simulink model "Final"  (R2023b)
settings: Solver=VariableStepAuto  StartTime=0.0  StopTime=150  FixedStep=0.05  RelTol=1e-5
undefined symbols (not defined in the file): adapt, ctrl, k_f, MRAC_on, Omega_prop_0, omegab_0, p_i_0, package_exist, par, pb_gate_cfg, q_0, robust_on, T_prop_0, task4_ground_z, UAV, UAV_pkg, v_i_0, vb_0
libraries: aerolibutil x3, sharedtransform x2, simulink_extras x2
settings Model: Creator=justs  LastModifiedBy=mghor
settings SolverCC: ZeroCrossAlgorithm=Adaptive
settings DataIOCC: SaveOutput=off  SignalLogging=off
settings OptimizationCC: ReuseModelBlockBuffer=off
settings DebuggingCC: IgnoredZcDiagnostic=none
settings ModelReferenceCC: EnableRefExpFcnMdlSchedulingChecks=on
settings ConfigComp: CovBoundaryAbsTol=1.0e-5

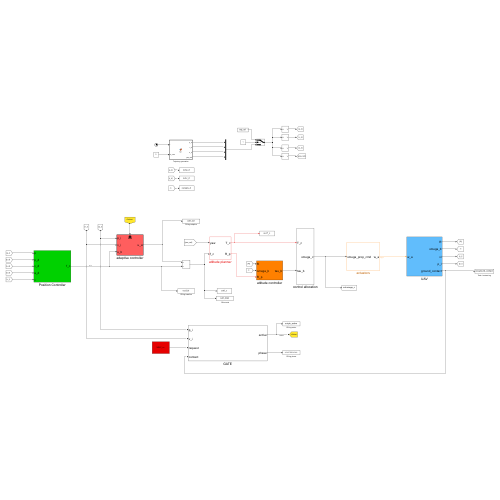
[thumbnail: Simulink's stored preview of the top-level diagram]
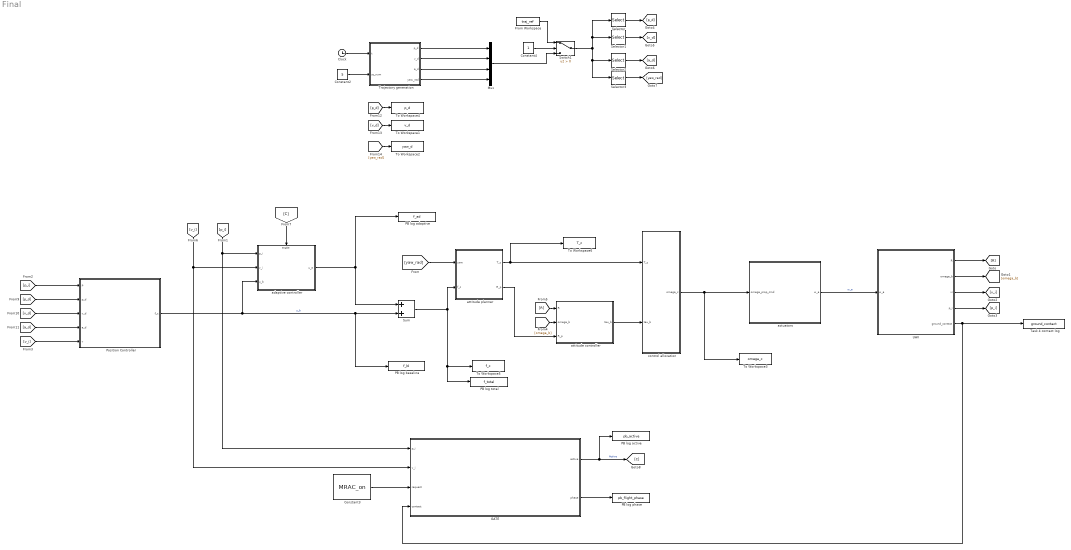
== system Final ==
  Clock : Clock
  Constant2 : Constant  Value=5
  Constant3 : Constant  Value=MRAC_on
  Constant4 : Constant
  From Workspace : FromWorkspace  VariableName=traj_ref  ZeroCross=off
  GATE : Subsystem
  Mux : Mux
  PB log active : ToWorkspace  VariableName=pb_active  SaveFormat=Timeseries  SampleTime=-1
  PB log adaptive : ToWorkspace  VariableName=f_ad  SaveFormat=Timeseries  SampleTime=-1
  PB log baseline : ToWorkspace  VariableName=f_bl  SaveFormat=Timeseries  SampleTime=-1
  PB log phase : ToWorkspace  VariableName=pb_flight_phase  SaveFormat=Timeseries  SampleTime=-1
  PB log total : ToWorkspace  VariableName=f_total  SaveFormat=Timeseries  SampleTime=-1
  Position Controller : Subsystem
  Selector : Selector  InputPortWidth=10  IndexOptions=Index vector (dialog)  Indices=[1 2 3]  OutputSizes=1
  Selector1 : Selector  InputPortWidth=10  IndexOptions=Index vector (dialog)  Indices=[4 5 6]  OutputSizes=1
  Selector2 : Selector  InputPortWidth=10  IndexOptions=Index vector (dialog)  Indices=[7 8 9]  OutputSizes=1
  Selector3 : Selector  InputPortWidth=10  IndexOptions=Index vector (dialog)  Indices=[10]  OutputSizes=1
  Sum : Sum
  Switch1 : Switch  Criteria=u2 > Threshold  SaturateOnIntegerOverflow=off  InputSameDT=off
  Task 4 contact log : ToWorkspace  VariableName=ground_contact  SaveFormat=Timeseries  SampleTime=-1
  To Workspace1 : ToWorkspace  VariableName=v_d  SaveFormat=Timeseries  SampleTime=-1
  To Workspace2 : ToWorkspace  VariableName=yaw_d  SaveFormat=Timeseries  SampleTime=-1
  To Workspace3 : ToWorkspace  VariableName=omega_c  SaveFormat=Timeseries  SampleTime=-1
  To Workspace4 : ToWorkspace  VariableName=p_d  SaveFormat=Timeseries  SampleTime=-1
  To Workspace5 : ToWorkspace  VariableName=f_c  SaveFormat=Timeseries  SampleTime=-1
  To Workspace6 : ToWorkspace  VariableName=T_c  SaveFormat=Timeseries  SampleTime=-1
  Trajectory generation : MATLAB Function  TreatAsAtomicUnit=on
  UAV : Subsystem
  actuators : Subsystem
  adaptive controller : Subsystem
  attitude controller : Subsystem
  attitude planner : Subsystem
  control allocation : Subsystem
  wires:
  Trajectory generation/2(v_d) -> Mux/2
  Trajectory generation/3(a_d) -> Mux/3
  Trajectory generation/1(p_d) -> Mux/1
  Clock/1 -> Trajectory generation/1(t)
  [p_i] -> Position Controller/1(p)
  [v_i] -> Position Controller/5(v)
  attitude planner/2(R_p) -> attitude controller/3(R_p)
  [omega_b] -> attitude controller/2(omega_b)
  [R] -> attitude controller/1(R)
  attitude planner/1(T_c) -> To Workspace6/1, control allocation/1(T_c)
  attitude controller/1(tau_b) -> control allocation/2(tau_b)
  control allocation/1(omega_c) -> To Workspace3/1, actuators/1(omega_prop_cmd)
  Trajectory generation/4(yaw_rad) -> Mux/4
  UAV/1(R) -> [R]
  UAV/2(omega_b) -> [omega_b]
  UAV/3(vi) -> [v_i]
  UAV/4(p_i) -> [p_i]
  Constant2/1 -> Trajectory generation/2(sc_num)
  actuators/1(w_a) -> UAV/1(w_a)  "w_a"
  [p_i] -> GATE/1(p_i), adaptive controller/1(p_i)
  [v_i] -> adaptive controller/2(v_i), GATE/2(v_i)
  Sum/1 -> PB log total/1, To Workspace5/1, attitude planner/2(f_c)
  Mux/1 -> Switch1/3
  Constant4/1 -> Switch1/2
  From Workspace/1 -> Switch1/1
  Selector/1 -> [p_d]
  Selector1/1 -> [v_d]
  Selector2/1 -> [a_d]
  Selector3/1 -> [yaw_rad]
  [yaw_rad] -> attitude planner/1(yaw)
  [p_d] -> Position Controller/2(p_d)
  [v_d] -> Position Controller/3(v_d)
  [a_d] -> Position Controller/4(a_d)
  [p_d] -> To Workspace4/1
  [v_d] -> To Workspace1/1
  [yaw_rad] -> To Workspace2/1
  Position Controller/1(f_c) -> Sum/2, PB log baseline/1, adaptive controller/3(u_b)  "u_b"
  adaptive controller/1(" u_a") -> PB log adaptive/1, Sum/1
  Switch1/1 -> Selector2/1, Selector3/1, Selector1/1, Selector/1
  UAV/5(ground_contact) -> GATE/4(contact), Task 4 contact log/1
  GATE/1(active) -> [C], PB log active/1  "Active"
  Constant3/1 -> GATE/3(request)
  GATE/2(phase) -> PB log phase/1
  [C] -> adaptive controller/Enable

== system Final/GATE ==
  p_i : Inport
  v_i : Inport  Port=2
  request : Inport  Port=3
  contact : Inport  Port=4
  PBMRAC enable : Subsystem  Variant=on
  active : Outport
  phase : Outport  Port=2
  wires:
  PBMRAC enable/1(active) -> active/1
  p_i/1 -> PBMRAC enable/1(p_i)
  request/1 -> PBMRAC enable/3(request)
  PBMRAC enable/2(phase) -> phase/1
  v_i/1 -> PBMRAC enable/2(v_i)
  contact/1 -> PBMRAC enable/4(contact)

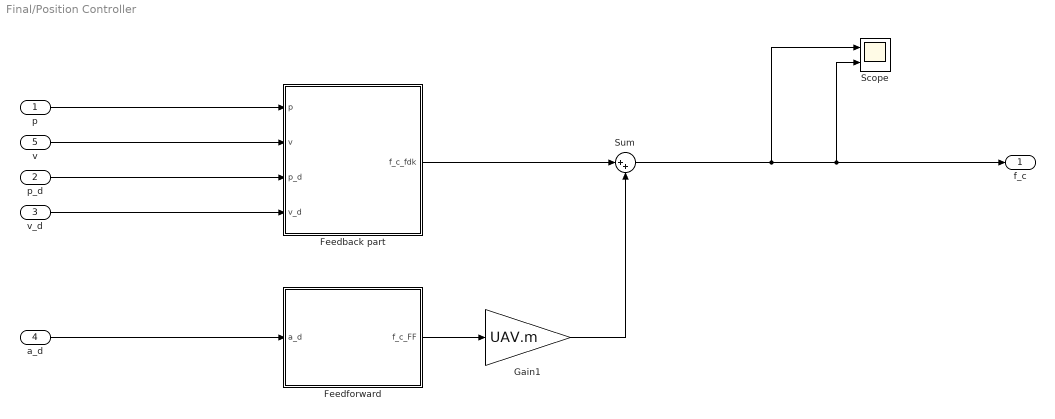
== system Final/Position Controller ==
  p : Inport
  p_d : Inport  Port=2
  v_d : Inport  Port=3
  a_d : Inport  Port=4
  v : Inport  Port=5
  Feedback part : Subsystem
  Feedforward : Subsystem
  Gain1 : Gain  Gain=UAV.m
  Scope : Scope  NumInputPorts=2
  Sum : Sum  Inputs=|++
  f_c : Outport
  wires:
  Feedback part/1(f_c_fdk) -> Sum/1
  v_d/1 -> Feedback part/4(v_d)
  Feedforward/1(f_c_FF) -> Gain1/1
  a_d/1 -> Feedforward/1(a_d)
  v/1 -> Feedback part/2(v)
  p_d/1 -> Feedback part/3(p_d)
  p/1 -> Feedback part/1(p)
  Sum/1 -> f_c/1, Scope/2, Scope/1
  Gain1/1 -> Sum/2

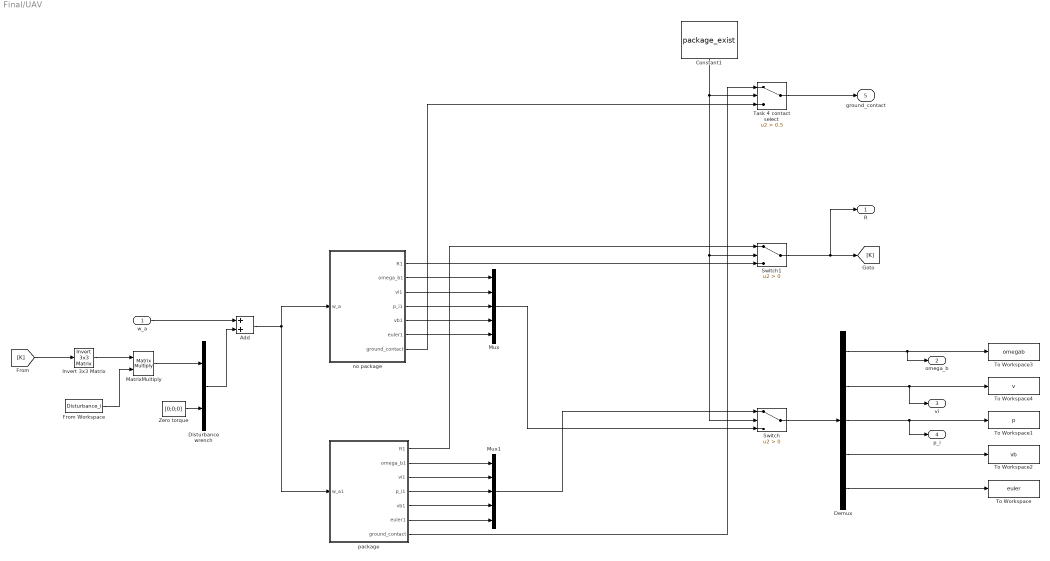
== system Final/UAV ==
  w_a : Inport
  Add : Sum
  Constant1 : Constant  Value=package_exist
  Demux : Demux  Outputs=5
  Disturbance wrench : Mux  Inputs=2
  From Workspace : FromWorkspace  VariableName=Disturbance_i
  Invert 3x3 Matrix : aerolibutil/Invert  3x3 Matrix
  MatrixMultiply : Product  Multiplication=Matrix(*)
  Mux : Mux  Inputs=5
  Mux1 : Mux  Inputs=5
  Switch : Switch  Criteria=u2 > Threshold  SaturateOnIntegerOverflow=off  InputSameDT=off
  Switch1 : Switch  Criteria=u2 > Threshold  SaturateOnIntegerOverflow=off  InputSameDT=off
  Task 4 contact select : Switch  Criteria=u2 > Threshold  Threshold=0.5  SaturateOnIntegerOverflow=off  InputSameDT=off
  To Workspace : ToWorkspace  VariableName=euler  SaveFormat=Timeseries  SampleTime=-1
  To Workspace1 : ToWorkspace  VariableName=p  SaveFormat=Timeseries  SampleTime=-1
  To Workspace2 : ToWorkspace  VariableName=vb  SaveFormat=Timeseries  SampleTime=-1
  To Workspace3 : ToWorkspace  VariableName=omegab  SaveFormat=Timeseries  SampleTime=-1
  To Workspace4 : ToWorkspace  VariableName=v  SaveFormat=Timeseries  SampleTime=-1
  Zero torque : Constant  Value=[0;0;0]
  no package : Subsystem
  package : Subsystem
  R : Outport
  omega_b : Outport  Port=2
  vi : Outport  Port=3
  p_i : Outport  Port=4
  ground_contact : Outport  Port=5
  wires:
  Constant1/1 -> Switch/2, Switch1/2, Task 4 contact select/2
  Mux1/1 -> Switch/1
  Mux/1 -> Switch/3
  no package/2(omega_b1) -> Mux/1
  no package/3(vi1) -> Mux/2
  no package/4(p_i1) -> Mux/3
  no package/5(vb1) -> Mux/4
  no package/6(euler1) -> Mux/5
  package/2(omega_b1) -> Mux1/1
  package/3(vi1) -> Mux1/2
  package/4(p_i1) -> Mux1/3
  package/5(vb1) -> Mux1/4
  package/6(euler1) -> Mux1/5
  Switch/1 -> Demux/1
  Demux/1 -> omega_b/1, To Workspace3/1
  Demux/2 -> To Workspace4/1, vi/1
  Demux/3 -> To Workspace1/1, p_i/1
  Demux/4 -> To Workspace2/1
  Demux/5 -> To Workspace/1
  no package/1(R1) -> Switch1/3
  package/1(R1) -> Switch1/1
  From Workspace/1 -> MatrixMultiply/2
  Switch1/1 -> R/1, [K]
  Zero torque/1 -> Disturbance wrench/2
  Disturbance wrench/1 -> Add/2
  Invert 3x3 Matrix/1 -> MatrixMultiply/1
  MatrixMultiply/1 -> Disturbance wrench/1
  w_a/1 -> Add/1
  Add/1 -> no package/1(w_a), package/1(w_a1)
  package/7(ground_contact) -> Task 4 contact select/1
  no package/7(ground_contact) -> Task 4 contact select/3
  Task 4 contact select/1 -> ground_contact/1
  [K] -> Invert 3x3 Matrix/1

== system Final/actuators ==
  omega_prop_cmd : Inport
  Constant1 : Constant  Value=UAV.F2
  Constant2 : Constant  Value=UAV.F1
  MatrixMultiply1 : Product  Inputs=3  Multiplication=Matrix(*)
  To Workspace1 : ToWorkspace  VariableName=w_a  SaveFormat=Timeseries  SampleTime=-1
  To Workspace6 : ToWorkspace  VariableName=T_out  SaveFormat=Timeseries  SampleTime=-1
  rotor_speed : Subsystem
  thrust : Subsystem
  w_a : Outport
  wires:
  rotor_speed/1(omega_prop) -> thrust/1(omega_prop)
  Constant2/1 -> MatrixMultiply1/1
  thrust/1(thrust) -> MatrixMultiply1/3, To Workspace6/1
  omega_prop_cmd/1 -> rotor_speed/1(omega_prop_cmd)
  MatrixMultiply1/1 -> w_a/1, To Workspace1/1
  Constant1/1 -> MatrixMultiply1/2

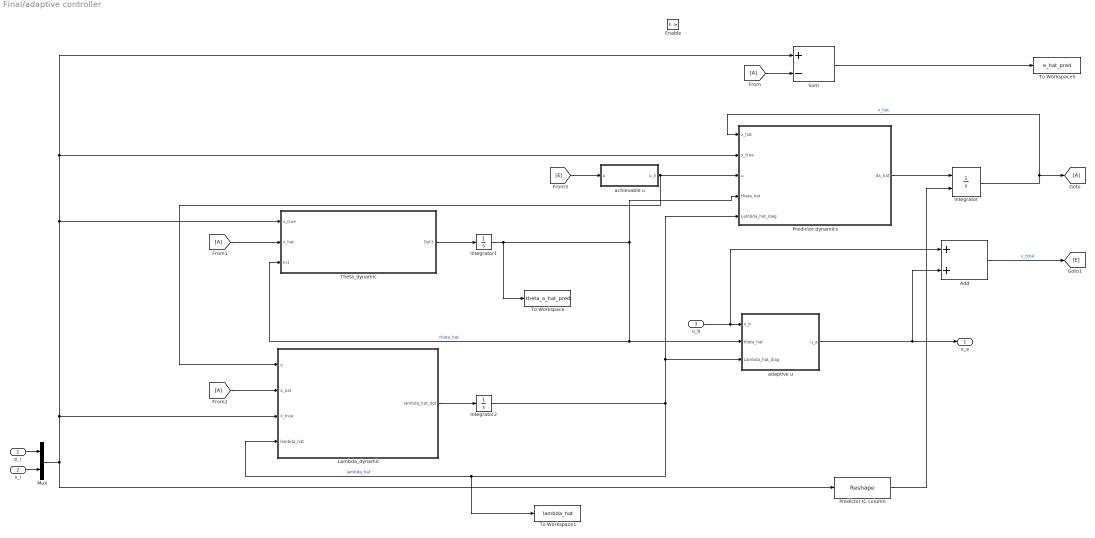
== system Final/adaptive controller ==
  p_i : Inport
  v_i : Inport  Port=2
  u_b : Inport  Port=3
  Enable : EnablePort  StatesWhenEnabling=reset
  Add : Sum
  From : From
  From1 : From
  From2 : From
  Goto : Goto
  Integrator : Integrator  InitialConditionSource=external  InitialCondition=[p_i_0; v_i_0]
  Integrator1 : Integrator  InitialCondition=[0; 0; 0]
  Integrator2 : Integrator  InitialCondition=[1;1;1]
  Lambda_dynamic : Subsystem
  Mux : Mux  Inputs=2
  Predictor IC column : Reshape  OutputDimensionality=Customize  OutputDimensions=[6 1]
  Predictor dynamics : MATLAB Function  TreatAsAtomicUnit=on
  Sum : Sum  Inputs=+-
  Theta_dynamic : Subsystem
  To Workspace : ToWorkspace  VariableName=theta_a_hat_pred  SaveFormat=Timeseries  SampleTime=-1
  To Workspace1 : ToWorkspace  VariableName=lambda_hat  SaveFormat=Timeseries  SampleTime=-1
  To Workspace5 : ToWorkspace  VariableName=e_hat_pred  SaveFormat=Timeseries  SampleTime=-1
  achievable u : MATLAB Function  TreatAsAtomicUnit=on
  adaptive u : MATLAB Function  TreatAsAtomicUnit=on
  " u_a" : Outport  OutputWhenDisabled=reset  InitialOutput=[0;0;0]
  wires:
  u_b/1 -> adaptive u/1(u_b), Add/1
  Add/1 -> [E]  "u_total"
  Integrator/1 -> Goto/1, Predictor dynamics/1(x_hat)  "x_hat"
  Integrator1/1 -> Predictor dynamics/4(theta_hat), Theta_dynamic/3(In1), adaptive u/2(theta_hat), To Workspace/1  "theta_hat"
  Integrator2/1 -> adaptive u/3(Lambda_hat_diag), Predictor dynamics/5(Lambda_hat_diag), To Workspace1/1, Lambda_dynamic/4(lambda_hat)  "lambda_hat"
  Mux/1 -> Sum/1, Predictor dynamics/2(x_true), Theta_dynamic/1(x_true), Lambda_dynamic/3(x_true), Predictor IC column/1
  adaptive u/1(u_a) -> " u_a"/1, Add/2
  From2/1 -> Lambda_dynamic/2(x_hat)
  From1/1 -> Theta_dynamic/2(x_hat)
  From/1 -> Sum/2
  Sum/1 -> To Workspace5/1
  Predictor dynamics/1(dx_hat) -> Integrator/1
  Theta_dynamic/1(Out1) -> Integrator1/1
  Lambda_dynamic/1(lambda_hat_dot) -> Integrator2/1
  p_i/1 -> Mux/1
  v_i/1 -> Mux/2
  achievable u/1(u_h) -> Predictor dynamics/3(u), Lambda_dynamic/1(u)
  Predictor IC column/1 -> Integrator/2
  [E] -> achievable u/1(u)

== system Final/attitude controller ==
  R : Inport
  omega_b : Inport  Port=2
  R_p : Inport  Port=3
  Gain : Gain  Gain=ctrl.Komega  Multiplication=Matrix(K*u)
  Saturation : Saturate  UpperLimit=1.2  LowerLimit=-1.2
  Scope : Scope  NumInputPorts=2
  Sum : Sum  Inputs=--
  e_R : MATLAB Function  TreatAsAtomicUnit=on
  tau_b : Outport
  wires:
  Saturation/1 -> Scope/2, tau_b/1
  e_R/1(e_R) -> Sum/1
  Sum/1 -> Saturation/1, Scope/1
  Gain/1 -> Sum/2
  R_p/1 -> e_R/2(R_d)
  R/1 -> e_R/1(R)
  omega_b/1 -> Gain/1

== system Final/attitude planner ==
  yaw : Inport
  f_c : Inport  Port=2
  MATLAB Function : MATLAB Function  TreatAsAtomicUnit=on
  T_c : Outport
  R_p : Outport  Port=2
  wires:
  yaw/1 -> MATLAB Function/1(yaw)
  f_c/1 -> MATLAB Function/2(f_c)
  MATLAB Function/1(T_c) -> T_c/1
  MATLAB Function/2(R_p) -> R_p/1

== system Final/control allocation ==
  T_c : Inport
  tau_b : Inport  Port=2
  Constant : Constant  Value=UAV.F2_pinv
  Constant1 : Constant  Value=k_f
  MATLAB Function : MATLAB Function  TreatAsAtomicUnit=on
  MATLAB Function1 : MATLAB Function  TreatAsAtomicUnit=on
  omega_c : Outport
  wires:
  T_c/1 -> MATLAB Function/1(T_c)
  tau_b/1 -> MATLAB Function/2(tau_b)
  MATLAB Function/1(Uc) -> MATLAB Function1/1(Uc)
  Constant/1 -> MATLAB Function/3(F2_pinv)
  MATLAB Function1/1(Omega_cmd) -> omega_c/1
  Constant1/1 -> MATLAB Function1/2(k_f)

== system Final/GATE/PBMRAC enable ==
  note: 1) Add Subsystem or Model blocks as valid variant choices.
      | 2) You cannot connect blocks at this level. At simulation, connectivity is automatically
      | determined, based on the active variant and port name matching.
  p_i : Inport
  v_i : Inport  Port=2
  request : Inport  Port=3
  contact : Inport  Port=4
  Direct : Subsystem  VariantControl=pb_flight_gate == 0
  Flight gate : Subsystem  VariantControl=pb_flight_gate == 1
  Subsystem1 : Subsystem  VariantControl=false
  active : Outport
  phase : Outport  Port=2

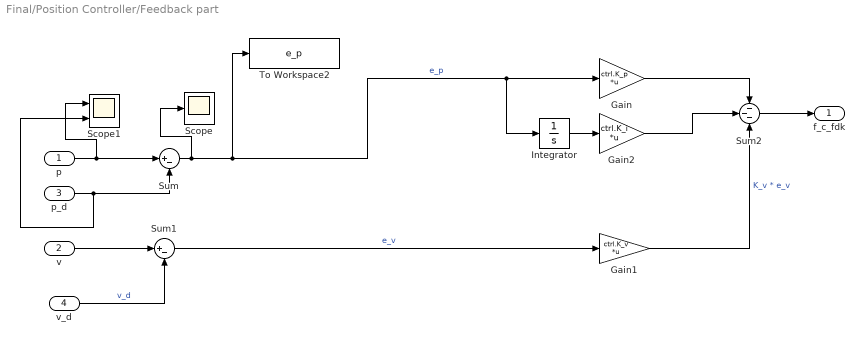
== system Final/Position Controller/Feedback part ==
  p : Inport
  v : Inport  Port=2
  p_d : Inport  Port=3
  v_d : Inport  Port=4
  Gain : Gain  Gain=ctrl.K_p  Multiplication=Matrix(K*u)
  Gain1 : Gain  Gain=ctrl.K_v  Multiplication=Matrix(K*u)
  Gain2 : Gain  Gain=ctrl.K_i  Multiplication=Matrix(K*u)
  Integrator : Integrator
  Scope : Scope
  Scope1 : Scope  NumInputPorts=2
  Sum : Sum  Inputs=|+-
  Sum1 : Sum  Inputs=|+-
  Sum2 : Sum  Inputs=---
  To Workspace2 : ToWorkspace  VariableName=e_p  SaveFormat=Timeseries  SampleTime=-1
  f_c_fdk : Outport
  wires:
  p_d/1 -> Scope1/2, Sum/2
  v/1 -> Sum1/1
  Sum1/1 -> Gain1/1  "e_v"
  v_d/1 -> Sum1/2  "v_d"
  p/1 -> Scope1/1, Sum/1
  Gain/1 -> Sum2/1
  Sum/1 -> Scope/1, To Workspace2/1, Integrator/1, Gain/1  "e_p"
  Integrator/1 -> Gain2/1
  Gain1/1 -> Sum2/3  "K_v * e_v"
  Sum2/1 -> f_c_fdk/1
  Gain2/1 -> Sum2/2

== system Final/Position Controller/Feedforward ==
  a_d : Inport
  Constant : Constant  Value=par.g*par.e_3
  Sum3 : Sum
  f_c_FF : Outport
  wires:
  Constant/1 -> Sum3/1
  a_d/1 -> Sum3/2
  Sum3/1 -> f_c_FF/1

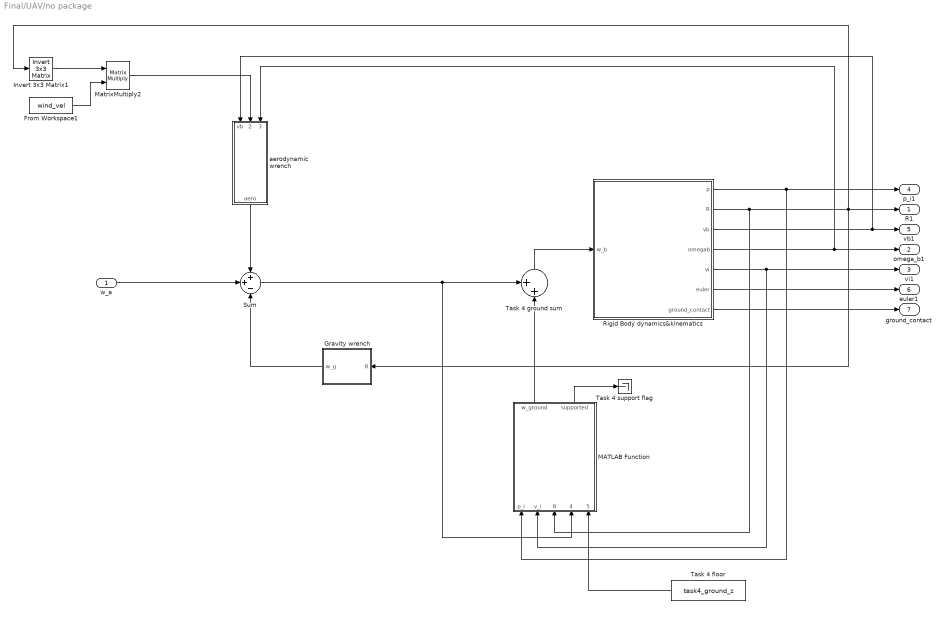
== system Final/UAV/no package ==
  w_a : Inport
  From Workspace1 : FromWorkspace  VariableName=wind_vel
  Gravity wrench : MATLAB Function  TreatAsAtomicUnit=on
  Invert 3x3 Matrix1 : aerolibutil/Invert  3x3 Matrix
  MATLAB Function : MATLAB Function  TreatAsAtomicUnit=on
  MatrixMultiply2 : Product  Multiplication=Matrix(*)
  "Rigid Body dynamics&kinematics " : Subsystem
  Sum : Sum  Inputs=++-
  Task 4 floor : Constant  Value=task4_ground_z
  Task 4 ground sum : Sum  Inputs=++|
  Task 4 support flag : Terminator
  aerodynamic wrench : Subsystem
  R1 : Outport
  omega_b1 : Outport  Port=2  PortDimensions=[3 1]
  vi1 : Outport  Port=3  PortDimensions=[3 1]
  p_i1 : Outport  Port=4  PortDimensions=[3 1]
  vb1 : Outport  Port=5  PortDimensions=[3 1]
  euler1 : Outport  Port=6  PortDimensions=[3 1]
  ground_contact : Outport  Port=7
  wires:
  "Rigid Body dynamics&kinematics "/4(omegab) -> omega_b1/1, aerodynamic wrench/3(omegab)
  "Rigid Body dynamics&kinematics "/3(vb) -> aerodynamic wrench/1(vb), vb1/1
  "Rigid Body dynamics&kinematics "/1(p) -> p_i1/1, MATLAB Function/1(p_i)
  "Rigid Body dynamics&kinematics "/5(vi) -> vi1/1, MATLAB Function/2(v_i)
  "Rigid Body dynamics&kinematics "/6(euler) -> euler1/1
  "Rigid Body dynamics&kinematics "/2(R) -> R1/1, Gravity wrench/1(R), Invert 3x3 Matrix1/1, MATLAB Function/3(R)
  aerodynamic wrench/1(aero) -> Sum/1
  Invert 3x3 Matrix1/1 -> MatrixMultiply2/1
  From Workspace1/1 -> MatrixMultiply2/2
  MatrixMultiply2/1 -> aerodynamic wrench/2(wind)
  Sum/1 -> MATLAB Function/4(w_free), Task 4 ground sum/1
  Task 4 ground sum/1 -> "Rigid Body dynamics&kinematics "/1(w_b)
  MATLAB Function/2(supported) -> Task 4 support flag/1
  "Rigid Body dynamics&kinematics "/7(ground_contact) -> ground_contact/1
  Task 4 floor/1 -> MATLAB Function/5(ground_z)
  w_a/1 -> Sum/2
  Gravity wrench/1(w_g) -> Sum/3
  MATLAB Function/1(w_ground) -> Task 4 ground sum/2

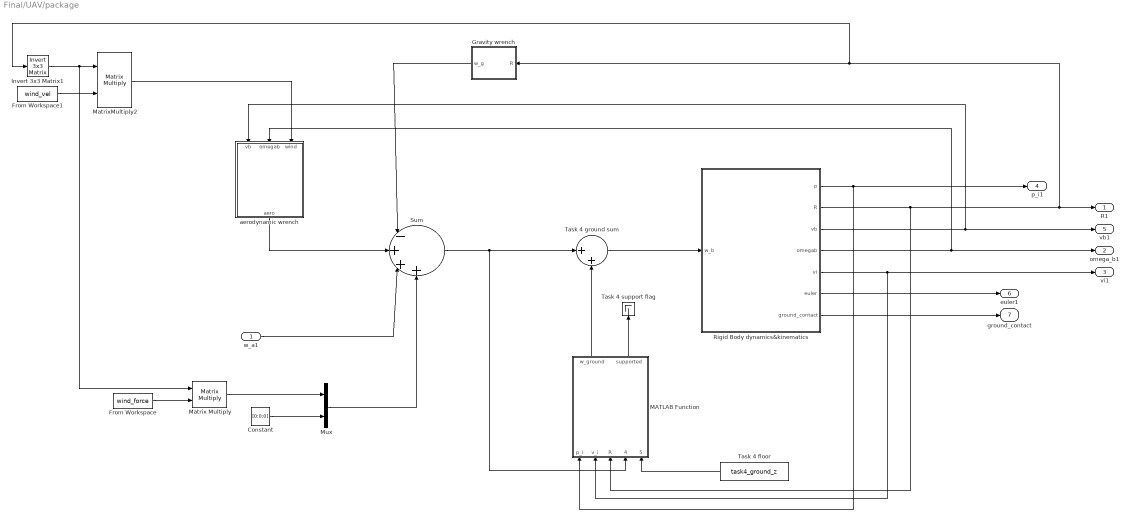
== system Final/UAV/package ==
  w_a1 : Inport
  Constant : Constant  Value=[0;0;0]
  From Workspace : FromWorkspace  VariableName=wind_force
  From Workspace1 : FromWorkspace  VariableName=wind_vel
  Gravity wrench : MATLAB Function  TreatAsAtomicUnit=on
  Invert 3x3 Matrix1 : aerolibutil/Invert  3x3 Matrix
  MATLAB Function : MATLAB Function  TreatAsAtomicUnit=on
  Matrix Multiply : Product  Multiplication=Matrix(*)
  MatrixMultiply2 : Product  Multiplication=Matrix(*)
  Mux : Mux  Inputs=2
  "Rigid Body dynamics&kinematics " : Subsystem
  Sum : Sum  Inputs=|-+++
  Task 4 floor : Constant  Value=task4_ground_z
  Task 4 ground sum : Sum  Inputs=|++
  Task 4 support flag : Terminator
  aerodynamic wrench : Subsystem
  R1 : Outport
  omega_b1 : Outport  Port=2  PortDimensions=[3 1]
  vi1 : Outport  Port=3  PortDimensions=[3 1]
  p_i1 : Outport  Port=4  PortDimensions=[3 1]
  vb1 : Outport  Port=5  PortDimensions=[3 1]
  euler1 : Outport  Port=6  PortDimensions=[3 1]
  ground_contact : Outport  Port=7
  wires:
  "Rigid Body dynamics&kinematics "/1(p) -> p_i1/1, MATLAB Function/1(p_i)
  "Rigid Body dynamics&kinematics "/5(vi) -> vi1/1, MATLAB Function/2(v_i)
  w_a1/1 -> Sum/3
  "Rigid Body dynamics&kinematics "/3(vb) -> vb1/1, aerodynamic wrench/1(vb)
  "Rigid Body dynamics&kinematics "/2(R) -> Invert 3x3 Matrix1/1, Gravity wrench/1(R), R1/1, MATLAB Function/3(R)
  "Rigid Body dynamics&kinematics "/4(omegab) -> omega_b1/1, aerodynamic wrench/2(omegab)
  "Rigid Body dynamics&kinematics "/6(euler) -> euler1/1
  aerodynamic wrench/1(aero) -> Sum/2
  Invert 3x3 Matrix1/1 -> Matrix Multiply/1, MatrixMultiply2/1
  From Workspace1/1 -> MatrixMultiply2/2
  MatrixMultiply2/1 -> aerodynamic wrench/3(wind)
  Gravity wrench/1(w_g) -> Sum/1
  From Workspace/1 -> Matrix Multiply/2
  Matrix Multiply/1 -> Mux/1
  Constant/1 -> Mux/2
  Mux/1 -> Sum/4
  Task 4 ground sum/1 -> "Rigid Body dynamics&kinematics "/1(w_b)
  MATLAB Function/2(supported) -> Task 4 support flag/1
  "Rigid Body dynamics&kinematics "/7(ground_contact) -> ground_contact/1
  Task 4 floor/1 -> MATLAB Function/5(ground_z)
  MATLAB Function/1(w_ground) -> Task 4 ground sum/2
  Sum/1 -> MATLAB Function/4(w_free), Task 4 ground sum/1

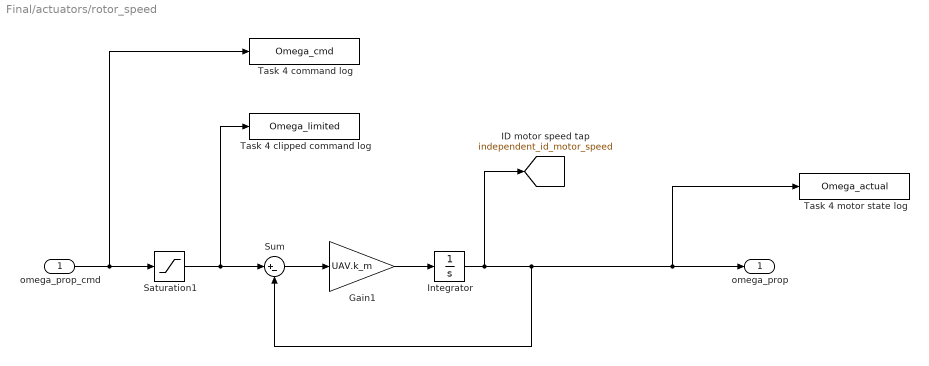
== system Final/actuators/rotor_speed ==
  omega_prop_cmd : Inport
  Gain1 : Gain  Gain=UAV.k_m
  Integrator : Integrator  InitialCondition=Omega_prop_0
  Saturation1 : Saturate  UpperLimit=UAV.Omega_max  LowerLimit=UAV.Omega_min
  Sum : Sum  Inputs=|+-
  Task 4 clipped command log : ToWorkspace  VariableName=Omega_limited  SaveFormat=Timeseries  SampleTime=-1
  Task 4 command log : ToWorkspace  VariableName=Omega_cmd  SaveFormat=Timeseries  SampleTime=-1
  Task 4 motor state log : ToWorkspace  VariableName=Omega_actual  SaveFormat=Timeseries  SampleTime=-1
  omega_prop : Outport
  tag scope: independent_id_motor_speed=global
  wires:
  omega_prop_cmd/1 -> Saturation1/1, Task 4 command log/1
  Sum/1 -> Gain1/1
  Gain1/1 -> Integrator/1
  Integrator/1 -> Task 4 motor state log/1, omega_prop/1, Sum/2, [independent_id_motor_speed]
  Saturation1/1 -> Sum/1, Task 4 clipped command log/1

== system Final/actuators/thrust ==
  omega_prop : Inport
  From Workspace : FromWorkspace  VariableName=lambda_sig
  Gain : Gain  Gain=k_f
  Product : Product
  Square : Math  Operator=square
  Transport Delay : TransportDelay  DelayTime=0.01  InitialOutput=T_prop_0
  thrust : Outport
  wires:
  omega_prop/1 -> Square/1
  Square/1 -> Gain/1
  Gain/1 -> Product/1
  From Workspace/1 -> Product/2
  Transport Delay/1 -> thrust/1
  Product/1 -> Transport Delay/1

== system Final/adaptive controller/Lambda_dynamic ==
  u : Inport
  x_hat : Inport  Port=2
  x_true : Inport  Port=3
  lambda_hat : Inport  Port=4
  Constant : Constant  Value=robust_on
  MATLAB Function : MATLAB Function  TreatAsAtomicUnit=on
  Switch : Switch  Criteria=u2 > Threshold  SaturateOnIntegerOverflow=off  InputSameDT=off
  lambda hat dot : MATLAB Function  TreatAsAtomicUnit=on
  lambda_hat_dot : Outport
  wires:
  x_true/1 -> lambda hat dot/2(x_true)
  lambda hat dot/1(d_Lambda_hat_diag) -> Switch/3, MATLAB Function/2(d_nom)
  Switch/1 -> lambda_hat_dot/1
  Constant/1 -> Switch/2
  MATLAB Function/1(d_proj) -> Switch/1
  x_hat/1 -> lambda hat dot/1(x_hat)
  u/1 -> lambda hat dot/3(u)
  lambda_hat/1 -> MATLAB Function/1(lambda_hat)

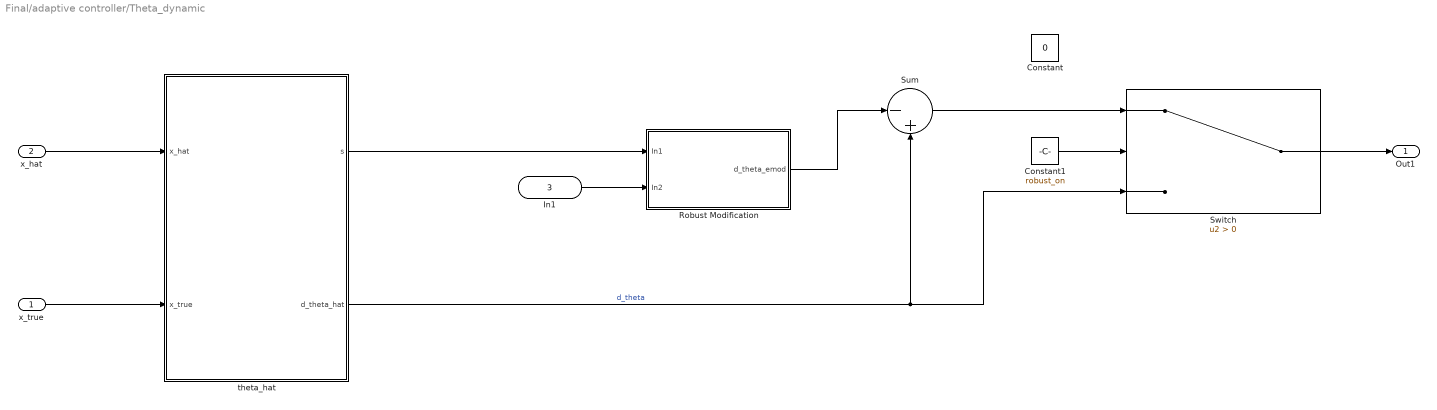
== system Final/adaptive controller/Theta_dynamic ==
  x_true : Inport
  x_hat : Inport  Port=2
  In1 : Inport  Port=3
  Constant : Constant  Value=0
  Constant1 : Constant  Value=robust_on
  Robust Modification : Subsystem
  Sum : Sum  Inputs=|-+
  Switch : Switch  Criteria=u2 > Threshold  SaturateOnIntegerOverflow=off  InputSameDT=off
  theta_hat : MATLAB Function  TreatAsAtomicUnit=on
  Out1 : Outport
  wires:
  x_true/1 -> theta_hat/2(x_true)
  x_hat/1 -> theta_hat/1(x_hat)
  Switch/1 -> Out1/1
  theta_hat/2(d_theta_hat) -> Sum/2, Switch/3  "d_theta"
  theta_hat/1(s) -> Robust Modification/1(In1)
  In1/1 -> Robust Modification/2(In2)
  Sum/1 -> Switch/1
  Robust Modification/1(d_theta_emod) -> Sum/1
  Constant1/1 -> Switch/2

== system Final/GATE/PBMRAC enable/Direct ==
  p_i : Inport
  v_i : Inport  Port=2
  request : Inport  Port=3
  contact : Inport  Port=4
  No phase : Constant  Value=0
  T1 : Terminator
  T2 : Terminator
  T4 : Terminator
  active : Outport
  phase : Outport  Port=2
  wires:
  p_i/1 -> T1/1
  v_i/1 -> T2/1
  contact/1 -> T4/1
  request/1 -> active/1
  No phase/1 -> phase/1

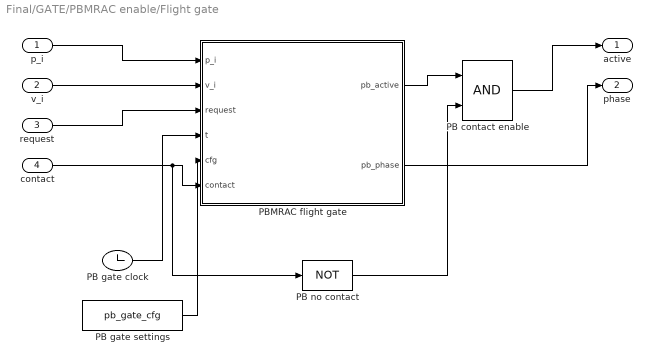
== system Final/GATE/PBMRAC enable/Flight gate ==
  p_i : Inport
  v_i : Inport  Port=2
  request : Inport  Port=3
  contact : Inport  Port=4
  PB contact enable : Logic  AllPortsSameDT=off  OutDataTypeStr=boolean
  PB gate clock : Clock
  PB gate settings : Constant  Value=pb_gate_cfg
  PB no contact : Logic  Operator=NOT  AllPortsSameDT=off  OutDataTypeStr=boolean
  PBMRAC flight gate : MATLAB Function  TreatAsAtomicUnit=on
  active : Outport
  phase : Outport  Port=2
  wires:
  p_i/1 -> PBMRAC flight gate/1(p_i)
  v_i/1 -> PBMRAC flight gate/2(v_i)
  request/1 -> PBMRAC flight gate/3(request)
  PB gate clock/1 -> PBMRAC flight gate/4(t)
  PB gate settings/1 -> PBMRAC flight gate/5(cfg)
  contact/1 -> PBMRAC flight gate/6(contact), PB no contact/1
  PBMRAC flight gate/1(pb_active) -> PB contact enable/1
  PB no contact/1 -> PB contact enable/2
  PB contact enable/1 -> active/1
  PBMRAC flight gate/2(pb_phase) -> phase/1

== system Final/GATE/PBMRAC enable/Subsystem1 ==
  In1 : Inport
  Out1 : Outport

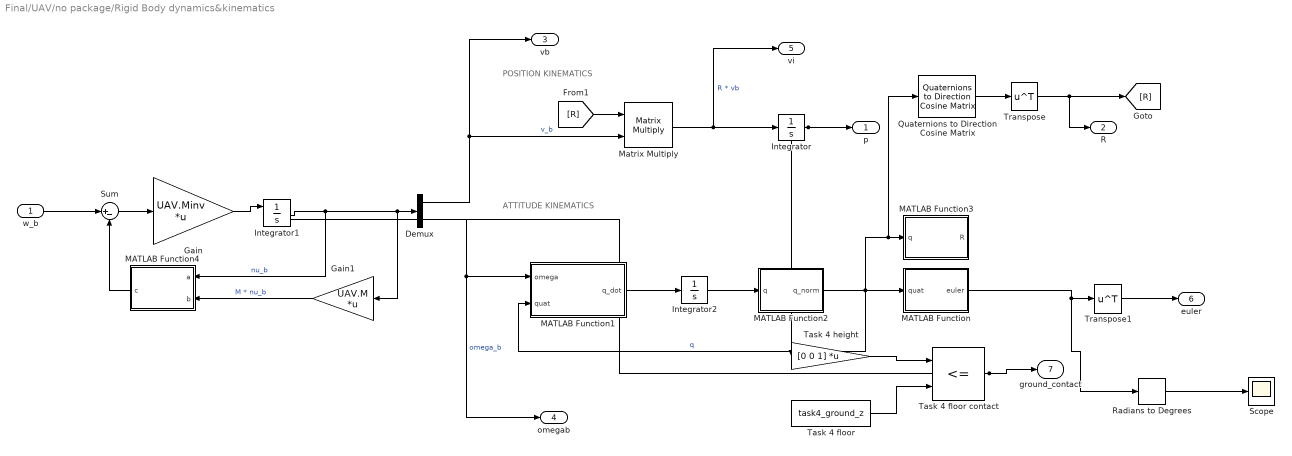
== system Final/UAV/no package/Rigid Body dynamics&kinematics  ==
  note: POSITION KINEMATICS
  note: ATTITUDE KINEMATICS
  w_b : Inport
  Demux : Demux  Outputs=2
  Gain : Gain  Gain=UAV.Minv  Multiplication=Matrix(K*u)
  Gain1 : Gain  Gain=UAV.M  Multiplication=Matrix(K*u)
  Integrator : Integrator  InitialCondition=p_i_0  LimitOutput=on  UpperSaturationLimit=[inf;inf;inf]  LowerSaturationLimit=[-inf;-inf;task4_ground_z]
  Integrator1 : Integrator  ExternalReset=rising  InitialCondition=[vb_0;omegab_0]
  Integrator2 : Integrator  InitialCondition=q_0
  MATLAB Function : MATLAB Function  TreatAsAtomicUnit=on
  MATLAB Function1 : MATLAB Function  TreatAsAtomicUnit=on
  MATLAB Function2 : MATLAB Function  TreatAsAtomicUnit=on
  MATLAB Function3 : MATLAB Function  TreatAsAtomicUnit=on
  MATLAB Function4 : MATLAB Function  TreatAsAtomicUnit=on
  Matrix Multiply : Product  Multiplication=Matrix(*)
  Quaternions to Direction Cosine Matrix : sharedtransform/Quaternions to  Direction Cosine Matrix  aMode=0
      settings: LibrarySourceBlock=|
      | aerolibtransform2/Quaternions to
      | Direction Cosine Matrix
  Radians to Degrees : simulink_extras/Transformations/Radians to Degrees
  Scope : Scope
  Sum : Sum  Inputs=|+-
  Task 4 floor : Constant  Value=task4_ground_z
  Task 4 floor contact : RelationalOperator  Operator=<=  OutDataTypeStr=boolean  RndMeth=Simplest  InputSameDT=off
  Task 4 height : Gain  Gain=[0 0 1]  Multiplication=Matrix(K*u)
  Transpose : Math  Operator=transpose
  Transpose1 : Math  Operator=transpose
  p : Outport  PortDimensions=[3 1]
  R : Outport  Port=2
  vb : Outport  Port=3
  omegab : Outport  Port=4
  vi : Outport  Port=5
  euler : Outport  Port=6
  ground_contact : Outport  Port=7
  wires:
  Radians to Degrees/1 -> Scope/1
  MATLAB Function/1(euler) -> Radians to Degrees/1, Transpose1/1
  Transpose/1 -> [R], R/1
  Quaternions to Direction Cosine Matrix/1 -> Transpose/1
  w_b/1 -> Sum/1
  MATLAB Function4/1(c) -> Sum/2
  Sum/1 -> Gain/1
  Gain1/1 -> MATLAB Function4/2(b)  "M * nu_b"
  Demux/2 -> MATLAB Function1/1(omega), omegab/1  "omega_b"
  Gain/1 -> Integrator1/1
  [R] -> Matrix Multiply/1
  Matrix Multiply/1 -> Integrator/1, vi/1  "R * vb"
  Integrator2/1 -> MATLAB Function2/1(q)
  Integrator1/1 -> MATLAB Function4/1(a), Gain1/1, Demux/1  "nu_b"
  Demux/1 -> Matrix Multiply/2, vb/1  "v_b"
  MATLAB Function2/1(q_norm) -> MATLAB Function/1(quat), MATLAB Function1/2(quat), MATLAB Function3/1(q), Quaternions to Direction Cosine Matrix/1  "q"
  MATLAB Function1/1(q_dot) -> Integrator2/1
  Integrator/1 -> p/1, Task 4 height/1
  Transpose1/1 -> euler/1
  Task 4 height/1 -> Task 4 floor contact/1
  Task 4 floor/1 -> Task 4 floor contact/2
  Task 4 floor contact/1 -> Integrator1/2, ground_contact/1

== system Final/UAV/no package/aerodynamic wrench ==
  vb : Inport
  wind : Inport  Port=2
  omegab : Inport  Port=3
  Constant5 : Constant  Value=-UAV.D
  MatrixMultiply3 : Product  Multiplication=Matrix(*)
  Minus : Sum  Inputs=+-
  Mux : Mux  Inputs=2
  Scope : Scope
  aero : Outport
  wires:
  MatrixMultiply3/1 -> aero/1  "aero"
  vb/1 -> Minus/1
  Constant5/1 -> MatrixMultiply3/1
  omegab/1 -> Mux/2
  Mux/1 -> MatrixMultiply3/2
  Minus/1 -> Scope/1, Mux/1
  wind/1 -> Minus/2

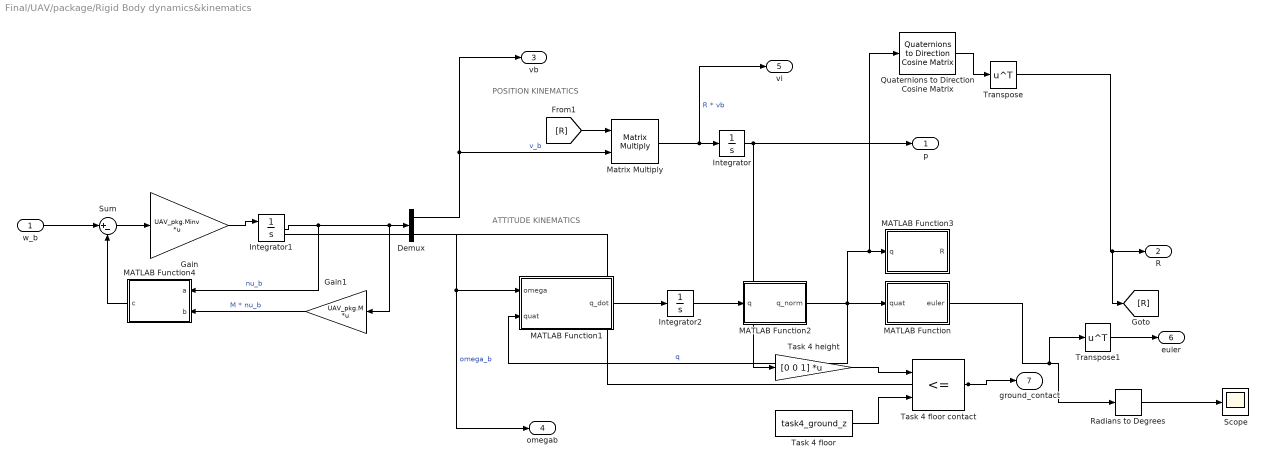
== system Final/UAV/package/Rigid Body dynamics&kinematics  ==
  note: ATTITUDE KINEMATICS
  note: POSITION KINEMATICS
  w_b : Inport
  Demux : Demux  Outputs=2
  Gain : Gain  Gain=UAV_pkg.Minv  Multiplication=Matrix(K*u)
  Gain1 : Gain  Gain=UAV_pkg.M  Multiplication=Matrix(K*u)
  Integrator : Integrator  InitialCondition=p_i_0  LimitOutput=on  UpperSaturationLimit=[inf;inf;inf]  LowerSaturationLimit=[-inf;-inf;task4_ground_z]
  Integrator1 : Integrator  ExternalReset=rising  InitialCondition=[vb_0;omegab_0]
  Integrator2 : Integrator  InitialCondition=q_0
  MATLAB Function : MATLAB Function  TreatAsAtomicUnit=on
  MATLAB Function1 : MATLAB Function  TreatAsAtomicUnit=on
  MATLAB Function2 : MATLAB Function  TreatAsAtomicUnit=on
  MATLAB Function3 : MATLAB Function  TreatAsAtomicUnit=on
  MATLAB Function4 : MATLAB Function  TreatAsAtomicUnit=on
  Matrix Multiply : Product  Multiplication=Matrix(*)
  Quaternions to Direction Cosine Matrix : sharedtransform/Quaternions to  Direction Cosine Matrix  aMode=0
      settings: LibrarySourceBlock=|
      | aerolibtransform2/Quaternions to
      | Direction Cosine Matrix
  Radians to Degrees : simulink_extras/Transformations/Radians to Degrees
  Scope : Scope
  Sum : Sum  Inputs=|+-
  Task 4 floor : Constant  Value=task4_ground_z
  Task 4 floor contact : RelationalOperator  Operator=<=  OutDataTypeStr=boolean  RndMeth=Simplest  InputSameDT=off
  Task 4 height : Gain  Gain=[0 0 1]  Multiplication=Matrix(K*u)
  Transpose : Math  Operator=transpose
  Transpose1 : Math  Operator=transpose
  p : Outport  PortDimensions=[3 1]
  R : Outport  Port=2
  vb : Outport  Port=3
  omegab : Outport  Port=4
  vi : Outport  Port=5
  euler : Outport  Port=6
  ground_contact : Outport  Port=7
  wires:
  Integrator/1 -> p/1, Task 4 height/1
  MATLAB Function1/1(q_dot) -> Integrator2/1
  MATLAB Function2/1(q_norm) -> Quaternions to Direction Cosine Matrix/1, MATLAB Function3/1(q), MATLAB Function1/2(quat), MATLAB Function/1(quat)  "q"
  Demux/1 -> vb/1, Matrix Multiply/2  "v_b"
  Integrator1/1 -> Demux/1, Gain1/1, MATLAB Function4/1(a)  "nu_b"
  Integrator2/1 -> MATLAB Function2/1(q)
  Matrix Multiply/1 -> vi/1, Integrator/1  "R * vb"
  [R] -> Matrix Multiply/1
  Gain/1 -> Integrator1/1
  Demux/2 -> omegab/1, MATLAB Function1/1(omega)  "omega_b"
  Gain1/1 -> MATLAB Function4/2(b)  "M * nu_b"
  Sum/1 -> Gain/1
  MATLAB Function4/1(c) -> Sum/2
  w_b/1 -> Sum/1
  Quaternions to Direction Cosine Matrix/1 -> Transpose/1
  Transpose/1 -> [R], R/1
  MATLAB Function/1(euler) -> Transpose1/1, Radians to Degrees/1
  Radians to Degrees/1 -> Scope/1
  Transpose1/1 -> euler/1
  Task 4 height/1 -> Task 4 floor contact/1
  Task 4 floor/1 -> Task 4 floor contact/2
  Task 4 floor contact/1 -> Integrator1/2, ground_contact/1

== system Final/UAV/package/aerodynamic wrench ==
  vb : Inport
  omegab : Inport  Port=2
  wind : Inport  Port=3
  Constant5 : Constant  Value=-UAV.D
  MatrixMultiply3 : Product  Multiplication=Matrix(*)
  Minus : Sum  Inputs=+-
  Mux : Mux  Inputs=2
  Scope : Scope
  aero : Outport
  wires:
  Mux/1 -> MatrixMultiply3/2
  omegab/1 -> Mux/2
  Constant5/1 -> MatrixMultiply3/1
  MatrixMultiply3/1 -> aero/1  "aero"
  vb/1 -> Minus/1
  Minus/1 -> Scope/1, Mux/1
  wind/1 -> Minus/2

== system Final/adaptive controller/Theta_dynamic/Robust Modification ==
  In1 : Inport
  In2 : Inport  Port=2
  Constant : Constant  Value=adapt.Gamma_theta
  Dot Product : DotProduct  OutDataTypeStr=Inherit: Inherit via internal rule
  Matrix Multiply : Product
  Matrix Multiply1 : Product  Multiplication=Matrix(*)
  Multiply : Gain  Gain=adapt.sigma_e
  Square Root : Sqrt
  d_theta_emod : Outport
  wires:
  Constant/1 -> Matrix Multiply1/1
  Matrix Multiply/1 -> d_theta_emod/1  "d_theta_emod"
  Multiply/1 -> Matrix Multiply/1
  In1/1 -> Dot Product/1, Dot Product/2
  Matrix Multiply1/1 -> Matrix Multiply/2
  Dot Product/1 -> Square Root/1
  Square Root/1 -> Multiply/1
  In2/1 -> Matrix Multiply1/2

== matlab function Final/adaptive controller/achievable u ==
  data: u input; u_h output
function u_h = achievable_u(u)
%ACHIEVABLE_U  The force the vehicle can actually receive (hedging).
%   The attitude planner caps the collective at T_MAX, so any command beyond
%   it is never applied. The predictor and the Lambda law are fed THIS force
%   instead of the commanded one, so saturation is not learned as a loss of
%   control effectiveness (which would drive Lambda_hat down, inflate u_a,
%   push the command further past the cap, and wind the adaptation up).
T_MAX = 22.9308;          % must match the cap in 'attitude planner'
n = norm(u);
if n > T_MAX
    u_h = u * (T_MAX / n);
else
    u_h = u;
end

== matlab function Final/UAV/no package/MATLAB Function ==
  data: p_i input; w_ground output; v_i input; R input; w_free input; supported output; ground_z input
function [w_ground, supported] = task4_ground_support(p_i, v_i, R, w_free, ground_z)
%TASK4_GROUND_SUPPORT Ideal sticking support on a flat landing surface.
%#codegen
% Used WITH the limited position state and the velocity impact reset added
% by upgrade_task4_contact. Wrench cancellation alone cannot stop a descent.
% R is body-to-inertial; w_free is the body wrench before ground reaction.
% This ideal support cancels force AND moment while resting on the floor.
% It has no compliance, bounce, finite friction cone, or landing-gear geometry.
% Tolerances (as in Antonio's original ground_support): without them,
% round-off in v_i = R*v_b makes v_i(3) flicker just above zero while the
% vehicle rests, the support drops for an instant, gravity adds a little
% downward velocity, and the support (which cancels force, not velocity)
% then freezes it: the vehicle "sinks" at a constant speed while its height
% is held at the floor.
z_tol = 1e-6;
v_tol = 1e-6;
w_ground = zeros(6,1);
supported = 0;
F_free_i = R*w_free(1:3);
if p_i(3) <= ground_z + z_tol && v_i(3) <= v_tol && F_free_i(3) <= 0
    w_ground = -w_free;
    supported = 1;
end
end

== matlab function Final/attitude controller/e_R ==
  data: R input; e_R output; R_d input; par parameter
function e_R = fcn(R,R_d,par)

k_R1 = par.k_R1;
k_R2 = par.k_R2;
k_R3 = par.k_R3;

e_1 = [1 0 0]';
e_2 = [0 1 0]';
e_3 = [0 0 1]';
R_e = R_d'*R; % transformation from body to desired frame coordinates

e_R = k_R1*cross(R_e'*e_1,e_1) + k_R2*cross(R_e'*e_2,e_2) + k_R3*cross(R_e'*e_3,e_3);

== matlab function Final/UAV/no package/Gravity wrench ==
  data: R input; w_g output; UAV parameter; par parameter
function w_g = fcn(R,UAV,par)

e_3 = par.e_3;
g = par.g;

w_g = g*[UAV.m*R'*e_3; UAV.S*R'*e_3];

== matlab function Final/UAV/package/MATLAB Function ==
  data: p_i input; w_ground output; v_i input; R input; w_free input; supported output; ground_z input
function [w_ground, supported] = task4_ground_support(p_i, v_i, R, w_free, ground_z)
%TASK4_GROUND_SUPPORT Ideal sticking support on a flat landing surface.
%#codegen
% Used WITH the limited position state and the velocity impact reset added
% by upgrade_task4_contact. Wrench cancellation alone cannot stop a descent.
% R is body-to-inertial; w_free is the body wrench before ground reaction.
% This ideal support cancels force AND moment while resting on the floor.
% It has no compliance, bounce, finite friction cone, or landing-gear geometry.
% Tolerances (as in Antonio's original ground_support): without them,
% round-off in v_i = R*v_b makes v_i(3) flicker just above zero while the
% vehicle rests, the support drops for an instant, gravity adds a little
% downward velocity, and the support (which cancels force, not velocity)
% then freezes it: the vehicle "sinks" at a constant speed while its height
% is held at the floor.
z_tol = 1e-6;
v_tol = 1e-6;
w_ground = zeros(6,1);
supported = 0;
F_free_i = R*w_free(1:3);
if p_i(3) <= ground_z + z_tol && v_i(3) <= v_tol && F_free_i(3) <= 0
    w_ground = -w_free;
    supported = 1;
end
end

== matlab function Final/GATE/PBMRAC enable/Flight gate/PBMRAC flight gate ==
  settings: updateMethod=DISCRETE  sampleTime=pb_gate_Ts
  data: p_i input; pb_active output; v_i input; request input; t input; cfg input; contact input; pb_phase output
function [pb_active, pb_phase] = task4_flight_gate(p_i, v_i, request, t, cfg, contact)
%TASK4_FLIGHT_GATE Measured-state supervisor for one delivery flight.
%#codegen
% Run this function at a DISCRETE sample time in Simulink, outside PBMRAC.
% cfg = [ground_z; enable_height; enable_vz; confirm_time].
% Phase: 0 waiting for lift-off, 1 airborne, 2 touchdown detected (latched).
% contact is the selected plant's floor-contact signal, not a height proxy.
% A separate continuous contact inhibit also disables the subsystem at impact,
% without waiting up to one supervisor sample for this latch to update.

persistent phase candidate_since
if isempty(phase)
    phase = 0;
    candidate_since = -1;
end

if request <= 0
    phase = 0;
    candidate_since = -1;
else
    height = p_i(3) - cfg(1);
    if phase == 0
        if contact <= 0.5 && height >= cfg(2) && v_i(3) >= cfg(3)
            if candidate_since < 0
                candidate_since = t;
            end
            if t - candidate_since >= cfg(4) - 1e-10
                phase = 1;
            end
        else
            candidate_since = -1;
        end
    elseif phase == 1
        % Stay active throughout descent, including the last millimetre.
        if contact > 0.5
            phase = 2;
        end
    end
end

pb_phase = phase;
pb_active = double(request > 0 && phase == 1);
end

== matlab function Final/adaptive controller/Predictor dynamics ==
  data: x_hat input; x_true input; u input; dx_hat output; theta_hat input; Lambda_hat_diag input; adapt parameter
function dx_hat = predictor(x_hat, x_true, u, theta_hat, Lambda_hat_diag, adapt)
    e_3 = [0; 0; 1];
    m   = adapt.m;
    g   = adapt.g;
    
    % Split states
    p_hat = x_hat(1:3);
    v_hat = x_hat(4:6);
    p_i   = x_true(1:3);
    v_i   = x_true(4:6);
    
    % Prediction error
    e_p_pos = p_i - p_hat;
    e_p_vel = v_i - v_hat;
    
    % Predictor dynamics
    % dp_hat = v_hat + L_p * (p_i - p_hat)
    % dv_hat = -g*e_3 + (1/m)*Lambda_hat*u + (1/m)*theta_hat + L_v*(v_i - v_hat)
    Lambda_hat = diag(Lambda_hat_diag);
    
    dp_hat = v_hat + adapt.L_p * e_p_pos;
    dv_hat =  + (1/m)*(Lambda_hat*u + theta_hat) + adapt.L_v * e_p_vel; %-g*e_3
    dv_hat = -g*e_3 + (1/m)*(Lambda_hat*u + theta_hat) + adapt.L_v * e_p_vel;
    dx_hat = [dp_hat; dv_hat];

== matlab function Final/adaptive controller/Theta_dynamic/theta_hat ==
  data: s output; x_hat input; d_theta_hat output; x_true input; adapt parameter
function [s,d_theta_hat] = update_theta(x_hat, x_true, adapt)
    % theta_dot_hat = Gamma_theta * (1/m) * P_v * (v_i - v_hat)
    % Since P is block-diagonal and we absorb (1/m)*P_v into Gamma_theta,
    % the effective update is:
    %   d_theta = Gamma_theta * (v_i - v_hat)
    v_hat = x_hat(4:6);
    v_i   = x_true(4:6);
    
    s = (v_i - v_hat) / adapt.m;
    d_theta_hat = adapt.Gamma_theta * s;

== matlab function Final/adaptive controller/Lambda_dynamic/lambda hat dot ==
  data: x_hat input; x_true input; u input; d_Lambda_hat_diag output size=[3 1]; adapt parameter
function d_Lambda_hat_diag = update_Lambda(x_hat, x_true, u, adapt)
    % For each diagonal element k:
    %   d_lambda_k = Gamma_lambda(k) * u(k) * (v_i_k - v_hat_k)
    v_hat = x_hat(4:6);
    v_i   = x_true(4:6);
    
    d_Lambda_hat_diag = adapt.Gamma_lambda .* u .* (v_i - v_hat) / adapt.m;
    %d_Lambda_hat_diag = adapt.Gamma_lambda .* u .* (v_i - v_hat) / adapt.m - adapt.sigma_lambda .* (Lambda_hat_diag - 1);

== matlab function Final/adaptive controller/adaptive u ==
  data: u_b input; u_a output; theta_hat input; Lambda_hat_diag input
function u_a = adaptive_input(u_b, theta_hat, Lambda_hat_diag)
    % u_a = (Lambda_hat^-1 - I) * u_b - Lambda_hat^-1 * theta_hat
    % With diagonal Lambda_hat, do it elementwise to avoid a 3x3 inverse.
    Lambda_inv = 1 ./ Lambda_hat_diag;   % 3x1
    
    u_a = (Lambda_inv - 1) .* u_b - Lambda_inv .* theta_hat;

== matlab function Final/UAV/package/Gravity wrench ==
  data: R input; w_g output; UAV_pkg parameter; par parameter
function w_g = fcn(R,UAV_pkg,par)

e_3 = par.e_3;
g = par.g;

w_g = g*[UAV_pkg.m*R'*e_3; UAV_pkg.S*R'*e_3];

== matlab function Final/UAV/package/Rigid Body dynamics&kinematics /MATLAB Function ==
  data: quat input; euler output
function euler = quatToEuler( quat )
%	Converts a quaternion vector to ZYX Euler angles (RPY)

euler = quat2eul(quat');

end

== matlab function Final/UAV/package/Rigid Body dynamics&kinematics /MATLAB Function1 ==
  data: omega input; quat input; q_dot output
 function q_dot = quat_kin(omega, quat)
%#codegen

eta = quat(1);
eps = quat(2:4);

W=[-eps';
   skew(eps) + eta*eye(3)];

q_dot = 0.5*W*omega;

end

function S=skew(s)
S=[0  -s(3)  s(2);
    s(3)   0 -s(1);
    -s(2)  s(1)  0];
end

== matlab function Final/UAV/no package/Rigid Body dynamics&kinematics /MATLAB Function ==
  data: quat input; euler output
function euler = quatToEuler( quat )
%	Converts a quaternion vector to ZYX Euler angles (RPY)

euler = quat2eul(quat');

end

== matlab function Final/UAV/package/Rigid Body dynamics&kinematics /MATLAB Function2 ==
  data: q input; q_norm output
function q_norm = quat_norm( q )

norm = sqrt( q(1)^2 + q(2)^2 + q(3)^2 + q(4)^2 );

q_norm = 1/norm * q;

== matlab function Final/UAV/package/Rigid Body dynamics&kinematics /MATLAB Function3 ==
  data: q input; R output
function R = fcn(q)

R = quat2rotm(q');

end

== matlab function Final/UAV/package/Rigid Body dynamics&kinematics /MATLAB Function4 ==
  data: a input; c output; b input
function c = cross_six(a,b)

a_v = a(1:3);
a_omega = a(4:6);

cross_six_var = [crossmat(a_omega), zeros(3,3);
             crossmat(a_v), crossmat(a_omega)] ;

c = cross_six_var*b;

end

function S=crossmat(s)
S=[0  -s(3)  s(2);
    s(3)   0 -s(1);
    -s(2)  s(1)  0];
end

== matlab function Final/UAV/no package/Rigid Body dynamics&kinematics /MATLAB Function1 ==
  data: omega input; quat input; q_dot output
 function q_dot = quat_kin(omega, quat)
%#codegen

eta = quat(1);
eps = quat(2:4);

W=[-eps';
   skew(eps) + eta*eye(3)];

q_dot = 0.5*W*omega;

end

function S=skew(s)
S=[0  -s(3)  s(2);
    s(3)   0 -s(1);
    -s(2)  s(1)  0];
end

== matlab function Final/UAV/no package/Rigid Body dynamics&kinematics /MATLAB Function2 ==
  data: q input; q_norm output
function q_norm = quat_norm( q )

norm = sqrt( q(1)^2 + q(2)^2 + q(3)^2 + q(4)^2 );

q_norm = 1/norm * q;

== matlab function Final/UAV/no package/Rigid Body dynamics&kinematics /MATLAB Function3 ==
  data: q input; R output
function R = fcn(q)

R = quat2rotm(q');

end

== matlab function Final/UAV/no package/Rigid Body dynamics&kinematics /MATLAB Function4 ==
  data: a input; c output; b input
function c = cross_six(a,b)

a_v = a(1:3);
a_omega = a(4:6);

cross_six_var = [crossmat(a_omega), zeros(3,3);
             crossmat(a_v), crossmat(a_omega)] ;

c = cross_six_var*b;

end

function S=crossmat(s)
S=[0  -s(3)  s(2);
    s(3)   0 -s(1);
    -s(2)  s(1)  0];
end

== matlab function Final/Trajectory generation ==
  data: p_d output; v_d output; a_d output; yaw_rad output; t input; sc_num input
function [p_d, v_d, a_d,yaw_rad ] = fcn(t,sc_num)
% Circular trajectory in the horizontal (x-y) plane at constant altitude,
% with yaw aligned to velocity direction (tangent to the circle).

% --- Trajectory parameters ---
    v_d = [0;
        0;
        0 ];
    p_d = [ 0*t;
        0;
        0 ];
    a_d=zeros(3,1);
    yaw_rad=0;
    return
if(sc_num==1)
    R     = 2;          % [m]   circle radius
    omega = 2;        % [rad/s] angular rate -> tangential speed = R*omega = 1 m/s
    z0    = 1;          % [m]   altitude (constant)
    phi0  = 0;          % [rad] initial phase

    % --- Phase angle ---
    phi = omega*t + phi0;

    % --- Position (3x1) ---
    p_d = [ R*cos(phi);
        R*sin(phi);
        z0 ];

    % --- Velocity (3x1) ---
    v_d = [-R*omega*sin(phi);
        R*omega*cos(phi);
        0 ];

    % --- Acceleration (3x1) ---
    a_d = [-R*omega^2*cos(phi);
        -R*omega^2*sin(phi);
        0 ];

    % --- Desired yaw: heading aligned with velocity vector ---
    yaw_rad = atan2(v_d(2), v_d(1));   % = phi + pi/2 for this circle
elseif sc_num==2
    if t < 5
        % Phase 1: hover at [0,0,1]
        p_d = [0; 0; 1];
        v_d = zeros(3,1); a_d = zeros(3,1);
        yaw_rad = 0;
    elseif t < 20
        % Phase 2: circle (R=2, omega=0.5)
        R_c = 2; omg = 0.5;
        phi = omg*(t-5);
        p_d = [R_c*cos(phi); R_c*sin(phi); 1];
        v_d = [-R_c*omg*sin(phi); R_c*omg*cos(phi); 0];
        a_d = [-R_c*omg^2*cos(phi); -R_c*omg^2*sin(phi); 0];
        yaw_rad = atan2(v_d(2), v_d(1));
    else
        % Phase 3: step to [2, 0, 1.5]
        p_d = [2; 0; 1.5];
        v_d = zeros(3,1); a_d = zeros(3,1);
        yaw_rad = 0;
    end
elseif sc_num==3
    p_d = [1; 0; 1];
    v_d = [0; 0; 0]; a_d = zeros(3,1);
    yaw_rad = 0;
elseif sc_num==5
% Helicoidal trajectory (reference-group comparison case)
    R_h   = 5;      % [m]     helix radius
    omg_h = 0.1;    % [rad/s] angular rate about vertical axis
    vz_h  = 0.5;    % [m/s]   constant climb rate
    z0_h  = 0;      % [m]     initial altitude

    phi = omg_h*t;

    p_d = [ R_h*cos(phi);
            R_h*sin(phi);
            z0_h + vz_h*t ];

    v_d = [-R_h*omg_h*sin(phi);
            R_h*omg_h*cos(phi);
            vz_h ];

    a_d = [-R_h*omg_h^2*cos(phi);
           -R_h*omg_h^2*sin(phi);
            0 ];

    yaw_rad = atan2(v_d(2), v_d(1));   % tangent-aligned heading
else
    A      = 1.5;     % [m] step amplitude
    z0     = 1;       % [m] base hover altitude
    T_step = 14;       % [s] duration of each half-step

    T_doub = 3*T_step;   % one doublet = +A, -A, 0
    T_two  = 2*T_doub;   % two doublets per block



    dx = 0; dy = 0; dz = 0;

    if t < T_two
        dx = doublet(t);                      % 2 doublets in x
    elseif t < 2*T_two
        dy = doublet(t - T_two);              % 2 doublets in y
    elseif t < 3*T_two
        dz = doublet(t - 2*T_two);            % 2 doublets in z
    elseif t < 4*T_two
        d = doublet(t - 3*T_two);             % 2 doublets all together
        dx = d; dy = d; dz = d;
    end

    p_d = [dx; dy; z0 + dz];
    v_d = [0; 0; 0];
    a_d = [0; 0; 0];
yaw_rate = 0.5;          % [rad/s] constant yaw rate
yaw_rad  = yaw_rate * t; % linearly increasing -> continuous rotation


end

    function s = doublet(tau)
        tau = mod(tau, T_doub);
        if tau < T_step
            s = A;
        elseif tau < 2*T_step
            s = -A;
        else
            s = 0;
        end
    end

end

== matlab function Final/attitude planner/MATLAB Function ==
  data: yaw input; f_c input; T_c output; R_p output
function [T_c, R_p]=fcn(yaw,f_c)

% Collective capped at 90% of the nominal maximum (6*k_f*Omega_max^2 = 25.48 N).
% Without headroom a saturated collective clips all six rotors, leaving no
% differential thrust for attitude torque (MC_run2 sample 236 flipped this way).
T_c=min(norm(f_c), 22.9308);

K_p=f_c/norm(f_c);

h_d=[cos(yaw);sin(yaw);0];

x = cross(K_p, h_d);
nx = norm(x);
if nx < 1e-6
    % fallback: use previous R_p or default
    J_p = [0; 1; 0];   % or hold last value
else
    J_p = x / nx;
end

I_p=cross(J_p,K_p);



R_p= [I_p, J_p, K_p];

== matlab function Final/control allocation/MATLAB Function ==
  data: T_c input; Uc output; tau_b input; F2_pinv input
function Uc = fcn(T_c, tau_b,F2_pinv )


Uc = F2_pinv  * [T_c; tau_b];

== matlab function Final/control allocation/MATLAB Function1 ==
  data: Uc input; Omega_cmd output; k_f input
function Omega_cmd = fcn(Uc,k_f)

T_cmd_safe = max(Uc, 0);              % no negative thrust
Omega_cmd  = sqrt(T_cmd_safe ./ k_f);   % then it's safe

== matlab function Final/adaptive controller/Lambda_dynamic/MATLAB Function ==
  data: lambda_hat input size=[3 1]; d_proj output size=[3 1]; d_nom input size=[3 1]; adapt parameter
function d_proj = projection_lambda(lambda_hat, d_nom,adapt)

center = adapt.lambda_proj_center;
r0 = adapt.lambda_proj_r0;
r1 = adapt.lambda_proj_r1;
d_proj = zeros(3,1);

den = r1^2 - r0^2;

for i = 1:3

    % Default: nominal adaptive law unchanged
    d_proj(i) = d_nom(i);

    z = lambda_hat(i) - center;

    f      = (z^2 - r0^2) / den;
    grad_f = 2*z / den;

    % Projection only acts outside the inner set
    % and only if adaptation points further outward.
    if (f > 0) && (d_nom(i)*grad_f > 0)

        alpha = f;

        if alpha > 1
            alpha = 1;
        elseif alpha < 0
            alpha = 0;
        end

        d_proj(i) = (1-alpha)*d_nom(i);
    end
end

end
